simulink model "baseline_pi"  (R2024b)
settings: Solver=FixedStepDiscrete  StartTime=0.0  StopTime=7200  FixedStep=0.5  RelTol=1e-3
libraries: slpidlib x1
settings Model: Creator=yuvrajsingh  LastModifiedBy=yuvrajsingh

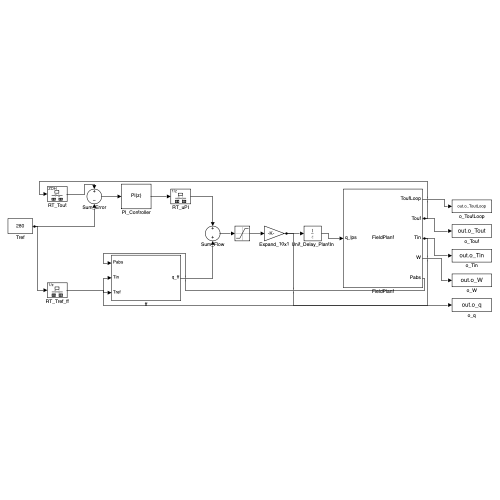
[thumbnail: Simulink's stored preview of the top-level diagram]
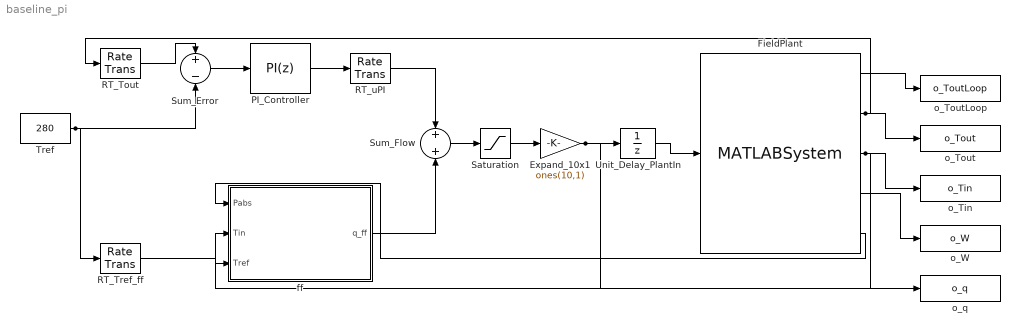
== system baseline_pi ==
  Expand_10x1 : Gain  Gain=ones(10,1)
  FieldPlant : MATLABSystem  System=FieldPlant
      mask Type: FieldPlant
      mask Display:
      | disp('FieldPlant');
      | port_label('input',1,'q_lps');
      | port_label('output',1,'ToutLoop');
      | port_label('output',2,'Tout');
      | port_label('output',3,'Tin');
      | port_label('output',4,'W');
      | port_label('output',5,'Pabs');
  PI_Controller : slpidlib/PID Controller  Controller=PI  Form=Parallel  TimeDomain=Discrete-time  UseExternalTs=off  SampleTime=5  IntegratorMethod=Forward Euler  FilterMethod=Forward Euler  ControllerParametersSource=internal  P=0.015475294  I=6.3100078e-05  UseKiTs=off  D=0  UseExternalDerivativeSource=off  N=100  UseFilter=on  TunerSelectOption=Transfer Function Based (PID Tuner App)  InitialConditionSource=internal  InitialConditionForIntegrator=0  InitialConditionForFilter=0  DifferentiatorICPrevScaledInput=0  ExternalReset=none  TrackingMode=off  Kt=1  LimitOutput=off  SatLimitsSource=internal  UpperSaturationLimit=inf  LowerSaturationLimit=-inf  LinearizeAsGain=off  AntiWindupMode=clamping  Kb=1  LimitIntegrator=off  UpperIntegratorSaturationLimit=inf  LowerIntegratorSaturationLimit=-inf  POutMin=[]  POutMax=[]  IOutMin=[]  IOutMax=[]  DOutMin=[]  DOutMax=[]  NOutMin=[]  NOutMax=[]  SumOutMin=[]  SumOutMax=[]  SaturationOutMin=[]  SaturationOutMax=[]  PParamMin=[]  PParamMax=[]  IParamMin=[]  IParamMax=[]  DParamMin=[]  DParamMax=[]  NParamMin=[]  NParamMax=[]  KbParamMin=[]  KbParamMax=[]  KtParamMin=[]  KtParamMax=[]  KbOutMin=[]  KbOutMax=[]  KtOutMin=[]  KtOutMax=[]  IntegratorOutMin=[]  IntegratorOutMax=[]  FilterOutMin=[]  FilterOutMax=[]  SumI1OutMin=[]  SumI1OutMax=[]  SumI2OutMin=[]  SumI2OutMax=[]  SumI3OutMin=[]  SumI3OutMax=[]  SumI4OutMin=[]  SumI4OutMax=[]  SumDOutMin=[]  SumDOutMax=[]  DifferentiatorOutMin=[]  DifferentiatorOutMax=[]  FilterDiffOutCoefMin=[]  FilterDiffOutCoefMax=[]  ReciprocalOutMin=[]  ReciprocalOutMax=[]  SumDenOutMin=[]  SumDenOutMax=[]  SumNumOutMin=[]  SumNumOutMax=[]  DivideOutMin=[]  DivideOutMax=[]  UdiffTsProdOutMin=[]  UdiffTsProdOutMax=[]  NTsProdOutMin=[]  NTsProdOutMax=[]  UintegralTsProdOutMin=[]  UintegralTsProdOutMax=[]  UngainTsProdOutMin=[]  UngainTsProdOutMax=[]  ClampingZeroOutDataTypeStr=Inherit: Inherit via back propagation  ClampingZeroOutMin=[]  ClampingZeroOutMax=[]  FilterDenConstantOutDataTypeStr=Inherit: Inherit via back propagation  FilterDenConstantOutMin=[]  FilterDenConstantOutMax=[]  PCopyOutDataTypeStr=Inherit: Inherit via back propagation  PCopyOutMin=[]  PCopyOutMax=[]  NCopyOutDataTypeStr=Inherit: Inherit via back propagation  NCopyOutMin=[]  NCopyOutMax=[]  IntegratorContinuousStateAttributes=''  IntegratorStateMustResolveToSignalObject=off  IntegratorRTWStateStorageClass=Auto  FilterContinuousStateAttributes=''  FilterStateMustResolveToSignalObject=off  FilterRTWStateStorageClass=Auto  ParallelPVariant=InternalParameters  IdealPVariant=Disabled  IVariant=InternalParameters  DVariant=Disabled  IntegratorVariant=Discrete  SatVariant=Disabled  AWVariant=Passthrough  PCopyVariant=Disabled  TRVariant=Disabled  FdbkBlocksVariant=Forward  IdealPFdbkVariant=Disabled  SatFdbkVariant=Disabled  DerivativeFilterVariant=Disabled  NVariant=Disabled  NCopyVariant=Disabled_SignalSpec  FilterICVariant=Disabled  IntegratorICVariant=InternalICs  ExternalResetVariant=Disabled  TRSumVariant=Passthrough  SumFdbkVariant=Disabled  SumVariant=Sum_PI  TsampFilterVariant=InternalTs  TsampNgainVariant=Passthrough  TsampIntegralVariant=Disabled_SignalSpec  ExternalSaturationOutDataTypeStr=Inherit: Same as second input  DerivativeSourceVariant=Disabled  PreIntVariant=InternalPreInt
      settings: LibrarySourceBlock=simulink/Discrete/Discrete PID Controller
  RT_Tout : RateTransition  OutPortSampleTime=5
  RT_Tref_ff : RateTransition  OutPortSampleTime=0.5
  RT_uPI : RateTransition  OutPortSampleTime=0.5
  Saturation : Saturate  UpperLimit=0.65  LowerLimit=0.2
  Sum_Error : Sum  Inputs=+-
  Sum_Flow : Sum
  Tref : Constant  Value=280  SampleTime=5
  Unit_Delay_PlantIn : UnitDelay  InitialCondition=0.5*ones(10,1)  SampleTime=0.5  HasFrameUpgradeWarning=on
  ff : Subsystem
  o_Tin : ToWorkspace  VariableName=o_Tin  SaveFormat=Structure With Time  SampleTime=0.5
  o_Tout : ToWorkspace  VariableName=o_Tout  SaveFormat=Structure With Time  SampleTime=0.5
  o_ToutLoop : ToWorkspace  VariableName=o_ToutLoop  SaveFormat=Structure With Time  SampleTime=0.5
  o_W : ToWorkspace  VariableName=o_W  SaveFormat=Structure With Time  SampleTime=0.5
  o_q : ToWorkspace  VariableName=o_q  SaveFormat=Structure With Time  SampleTime=0.5
  wires:
  FieldPlant/2 -> RT_Tout/1, o_Tout/1
  RT_Tout/1 -> Sum_Error/1
  Tref/1 -> Sum_Error/2, RT_Tref_ff/1
  Sum_Error/1 -> PI_Controller/1
  PI_Controller/1 -> RT_uPI/1
  RT_uPI/1 -> Sum_Flow/1
  FieldPlant/5 -> ff/1(Pabs)
  FieldPlant/3 -> ff/2(Tin), o_Tin/1
  RT_Tref_ff/1 -> ff/3(Tref)
  ff/1(q_ff) -> Sum_Flow/2
  Sum_Flow/1 -> Saturation/1
  Saturation/1 -> Expand_10x1/1
  Expand_10x1/1 -> Unit_Delay_PlantIn/1, o_q/1
  Unit_Delay_PlantIn/1 -> FieldPlant/1
  FieldPlant/1 -> o_ToutLoop/1
  FieldPlant/4 -> o_W/1

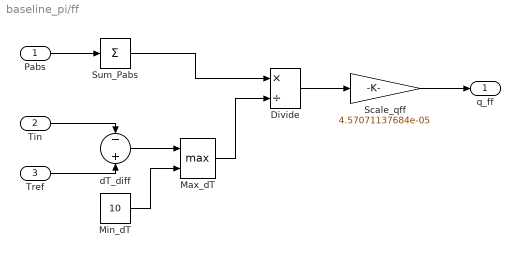
== system baseline_pi/ff ==
  Pabs : Inport
  Tin : Inport  Port=2
  Tref : Inport  Port=3
  Divide : Product  Inputs=*/
  Max_dT : MinMax  Function=max  Inputs=2
  Min_dT : Constant  Value=10
  Scale_qff : Gain  Gain=4.57071137684e-05
  Sum_Pabs : Sum  Inputs=+
  dT_diff : Sum  Inputs=-+
  q_ff : Outport
  wires:
  Pabs/1 -> Sum_Pabs/1
  Tin/1 -> dT_diff/1
  Tref/1 -> dT_diff/2
  dT_diff/1 -> Max_dT/1
  Min_dT/1 -> Max_dT/2
  Sum_Pabs/1 -> Divide/1
  Max_dT/1 -> Divide/2
  Divide/1 -> Scale_qff/1
  Scale_qff/1 -> q_ff/1
